simulink model "single_phase_ttype_inverter"  (R2026a)
settings: Solver=ode23tb  StopTime=simlength  FixedStep=tc  MaxStep=glb_time.tc
values from neighbouring files (symbols this model uses):
  afe_ctrl = param.afe.ctrl    [init_model.m]
  afe_pwm_phase_shift_mod1 = param.afe.behav.pwm_phase_shift_mod1    [init_model.m]
  DThs_init = param.thermal.DThs_init    [init_model.m]
  filters = param.ctrl.filters    [init_model.m]
  frt_data = param.frt.data    [init_model.m]
  glb_time = param.glb_time    [init_model.m]
  grid_emu = param.grid.emu    [init_model.m]
  kepsilon = param.spinv.kepsilon    [init_model.m]
  kp_align = param.ctrl.kp_align    [init_model.m]
  lim_down_align = param.ctrl.lim_down_align    [init_model.m]
  lim_up_align = param.ctrl.lim_up_align    [init_model.m]
  mavarage_filter_frequency_base_order = param.ctrl.mavarage_filter_frequency_base_order    [init_model.m]
  omega_set = param.spinv.omega_set    [init_model.m]
  single_phase_inverter_ctrl = param.spinv.ctrl    [init_model.m]
  Tambient = param.thermal.Tambient    [init_model.m]
  time_aux_power_supply_fault = param.sim.time_aux_power_supply_fault    [init_model.m]
  time_step_ref_1 = param.spinv.ref.time_step_ref_1    [init_model.m]
  time_step_ref_2 = param.spinv.ref.time_step_ref_2    [init_model.m]
  time_step_ref_3 = param.spinv.ref.time_step_ref_3    [init_model.m]
undefined symbols (not defined in the file or in its folder): delta_fht1, hwdata, ki_align, Ld_fht1, magnitude, omega_fht1, ts_inv, Vac_FS, Vdc_nom, Xbez
libraries: fl_lib x61, nesl_utility x39, moving_average_filter x11, moving_average_filter_cc x8, discrete_time_low_pass_filter x4, sl_discontinuities x3, single_phase_transformer_lib x3, linear_double_integrator_observer_ccaller x2, phase_shift_filter_ccaller x2, threephase_inductor_lib x1, dclink_for_two_levels x1, three_phase_pwm_modulator x1
(part 3 of 9)

== system single_phase_ttype_inverter/single_phase_inverter/single phase inverter control/acquisition_and_scaling_grid_voltage_ac ==
  in : Inport
  1/Ti5 : Gain  Gain=1/grid_emu.u2bez  SaturateOnIntegerOverflow=on  OutDataTypeStr=Inherit: Same as input  ParamDataTypeStr=Inherit: Same as input
  Quantizer : Quantizer  QuantizationInterval=adc12_quantization
  out : Outport
  wires:
  Quantizer/1 -> out/1
  1/Ti5/1 -> Quantizer/1
  in/1 -> 1/Ti5/1

== system single_phase_ttype_inverter/single_phase_inverter/single phase inverter control/acquisition_and_scaling_voltage ==
  in : Inport
  1/Ti5 : Gain  Gain=1/hwdata.single_phase_inverter.ubez  SaturateOnIntegerOverflow=on  OutDataTypeStr=Inherit: Same as input  ParamDataTypeStr=Inherit: Same as input
  Quantizer : Quantizer  QuantizationInterval=adc12_quantization
  pwm filtering for measure : cstblocks_lti/LTI System  sys=sogi.flt.beta  IC=[]  PadeOrder=0
  out : Outport
  wires:
  in/1 -> 1/Ti5/1
  pwm filtering for measure/1 -> Quantizer/1
  1/Ti5/1 -> pwm filtering for measure/1
  Quantizer/1 -> out/1

== system single_phase_ttype_inverter/single_phase_inverter/single phase inverter control/inverter_current_output_pu_reference ==
  Gain : Gain
  Rate Limiter : RateLimiter  RisingSlewLimit=hwdata.single_phase_inverter.ibez  FallingSlewLimit=-hwdata.single_phase_inverter.ibez  SampleTimeMode=inherited
  Sum : Sum  Inputs=+++
  i_out_inverter_reference_step1 : Step  Time=time_step_ref_1  FinalValue=iph_grid_pu_ref_1  SampleTime=0
  i_out_inverter_reference_step2 : Step  Time=time_step_ref_2  FinalValue=iph_grid_pu_ref_2  SampleTime=0
  i_out_inverter_reference_step3 : Step  Time=time_step_ref_3  FinalValue=iph_grid_pu_ref_3  SampleTime=0
  inverter_current_output_pu_reference : Outport
  wires:
  Rate Limiter/1 -> Gain/1
  Sum/1 -> Rate Limiter/1
  Gain/1 -> inverter_current_output_pu_reference/1
  i_out_inverter_reference_step1/1 -> Sum/2
  i_out_inverter_reference_step2/1 -> Sum/3
  i_out_inverter_reference_step3/1 -> Sum/1

== system single_phase_ttype_inverter/single_phase_inverter/single phase inverter control/pwm modulator ==
  vout : Inport
  Constant : Constant  Value=0
  single_phase_three_levels_PWM_generator_with_global_TRGO : single_phase_three_levels_PWM_modulator/single_phase_three_levels_PWM_generator_with_global_TRGO  f=glb_time.fPWM_INV  m_up=1  m_low=-1  dead_time=glb_time.dead_time_INV  pos_cmd_gate=15  neg_cmd_gate=-10  polarity=1  tc=glb_time.tc  double_sampling=0
  gate_cmds : Outport
  tag scope: TRGO_INV_1=global
  wires:
  vout/1 -> single_phase_three_levels_PWM_generator_with_global_TRGO/3
  Constant/1 -> single_phase_three_levels_PWM_generator_with_global_TRGO/2
  single_phase_three_levels_PWM_generator_with_global_TRGO/2 -> gate_cmds/1
  single_phase_three_levels_PWM_generator_with_global_TRGO/1 -> [TRGO_INV_1]
  [local_time_inverter] -> single_phase_three_levels_PWM_generator_with_global_TRGO/1

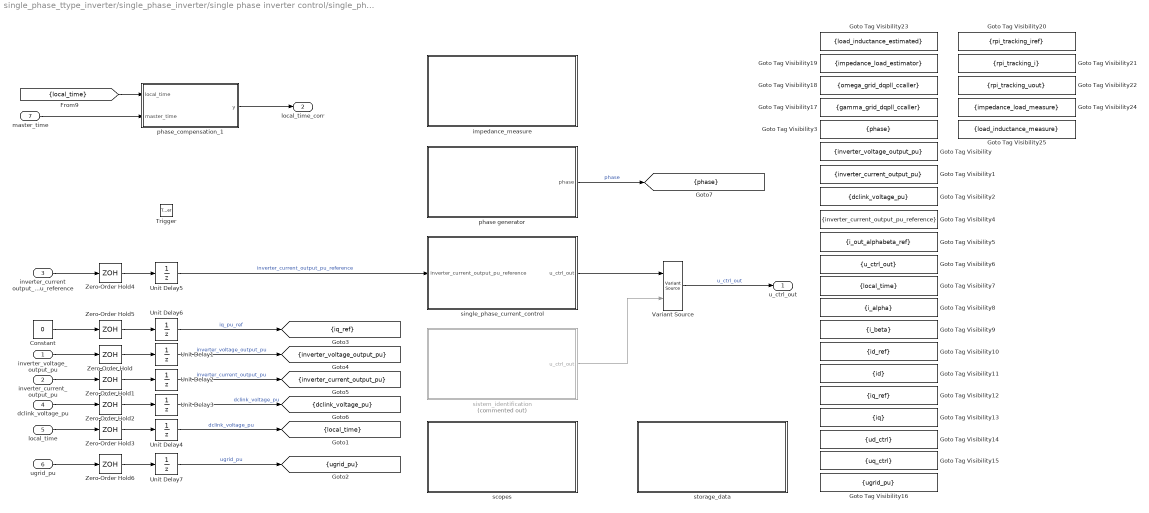
== system single_phase_ttype_inverter/single_phase_inverter/single phase inverter control/single_phase_inverter_ctrl ==
  inverter_voltage_output_pu : Inport
  inverter_current_output_pu : Inport  Port=2
  inverter_current output_pu_reference : Inport  Port=3
  dclink_voltage_pu : Inport  Port=4
  local_time : Inport  Port=5
  ugrid_pu : Inport  Port=6
  master_time : Inport  Port=7
  Trigger : TriggerPort  VariantControl=(inherit)  PortDimensions=1
  Constant : Constant  Value=0
  Goto Tag Visibility : GotoTagVisibility  GotoTag=inverter_voltage_output_pu
  Goto Tag Visibility1 : GotoTagVisibility  GotoTag=inverter_current_output_pu
  Goto Tag Visibility10 : GotoTagVisibility  GotoTag=id_ref
  Goto Tag Visibility11 : GotoTagVisibility  GotoTag=id
  Goto Tag Visibility12 : GotoTagVisibility  GotoTag=iq_ref
  Goto Tag Visibility13 : GotoTagVisibility  GotoTag=iq
  Goto Tag Visibility14 : GotoTagVisibility  GotoTag=ud_ctrl
  Goto Tag Visibility15 : GotoTagVisibility  GotoTag=uq_ctrl
  Goto Tag Visibility16 : GotoTagVisibility  GotoTag=ugrid_pu
  Goto Tag Visibility17 : GotoTagVisibility  GotoTag=gamma_grid_dqpll_ccaller
  Goto Tag Visibility18 : GotoTagVisibility  GotoTag=omega_grid_dqpll_ccaller
  Goto Tag Visibility19 : GotoTagVisibility  GotoTag=impedance_load_estimator
  Goto Tag Visibility2 : GotoTagVisibility  GotoTag=dclink_voltage_pu
  Goto Tag Visibility20 : GotoTagVisibility  GotoTag=rpi_tracking_iref
  Goto Tag Visibility21 : GotoTagVisibility  GotoTag=rpi_tracking_i
  Goto Tag Visibility22 : GotoTagVisibility  GotoTag=rpi_tracking_uout
  Goto Tag Visibility23 : GotoTagVisibility  GotoTag=load_inductance_estimated
  Goto Tag Visibility24 : GotoTagVisibility  GotoTag=impedance_load_measure
  Goto Tag Visibility25 : GotoTagVisibility  GotoTag=load_inductance_measure
  Goto Tag Visibility3 : GotoTagVisibility  GotoTag=phase
  Goto Tag Visibility4 : GotoTagVisibility  GotoTag=inverter_current_output_pu_reference
  Goto Tag Visibility5 : GotoTagVisibility  GotoTag=i_out_alphabeta_ref
  Goto Tag Visibility6 : GotoTagVisibility  GotoTag=u_ctrl_out
  Goto Tag Visibility7 : GotoTagVisibility  GotoTag=local_time
  Goto Tag Visibility8 : GotoTagVisibility  GotoTag=i_alpha
  Goto Tag Visibility9 : GotoTagVisibility  GotoTag=i_beta
  Unit Delay{1..7} (7 alike) : UnitDelay  SampleTime=-1
  Variant Source : VariantSource  VariantControls={system_identification_enable == 0, system_identification_enable == 1}
  Zero-Order Hold{,1..6} (7 alike) : ZeroOrderHold  SampleTime=-1
  impedance_measure : Subsystem
  phase generator : Subsystem
  phase_compensation_1 : Subsystem
  scopes : Subsystem
  single_phase_current_control : Subsystem
  sistem_identification : Subsystem  Commented=on
  storage_data : Subsystem
  u_ctrl_out : Outport
  local_time_corr : Outport  Port=2
  tag scope: dclink_voltage_pu=scoped, inverter_current_output_pu=scoped, inverter_voltage_output_pu=scoped, iq_ref=scoped, local_time=scoped, phase=scoped, ugrid_pu=scoped
  wires:
  inverter_voltage_output_pu/1 -> Zero-Order Hold/1
  inverter_current_output_pu/1 -> Zero-Order Hold1/1
  dclink_voltage_pu/1 -> Zero-Order Hold2/1
  Unit Delay1/1 -> [inverter_voltage_output_pu]  "inverter_voltage_output_pu"
  Unit Delay2/1 -> [inverter_current_output_pu]  "inverter_current_output_pu"
  Unit Delay3/1 -> [dclink_voltage_pu]  "dclink_voltage_pu"
  phase generator/1(phase) -> [phase]  "phase"
  inverter_current output_pu_reference/1 -> Zero-Order Hold4/1
  single_phase_current_control/1(u_ctrl_out) -> Variant Source/1
  Variant Source/1 -> u_ctrl_out/1  "u_ctrl_out"
  sistem_identification/1(u_ctrl_out) -> Variant Source/2
  Zero-Order Hold/1 -> Unit Delay1/1
  Zero-Order Hold1/1 -> Unit Delay2/1
  Zero-Order Hold2/1 -> Unit Delay3/1
  Zero-Order Hold3/1 -> Unit Delay4/1
  Unit Delay4/1 -> [local_time]  "dclink_voltage_pu"
  local_time/1 -> Zero-Order Hold3/1
  Zero-Order Hold4/1 -> Unit Delay5/1
  Unit Delay5/1 -> single_phase_current_control/1(inverter_current_output_pu_reference)  "inverter_current_output_pu_reference"
  Constant/1 -> Zero-Order Hold5/1
  Zero-Order Hold5/1 -> Unit Delay6/1
  Unit Delay6/1 -> [iq_ref]  "iq_pu_ref"
  ugrid_pu/1 -> Zero-Order Hold6/1
  Zero-Order Hold6/1 -> Unit Delay7/1
  Unit Delay7/1 -> [ugrid_pu]  "ugrid_pu"
  [local_time] -> phase_compensation_1/1(local_time)
  phase_compensation_1/1(y) -> local_time_corr/1
  master_time/1 -> phase_compensation_1/2(master_time)

== system single_phase_ttype_inverter/afe/AFE_control/afe_control/FRT-VDE4110 ==
  FRT-Detection : Subsystem
  FRT-PosNegReactiveCurrentReferences : Subsystem
  frt_detection_output : Scope  NumInputPorts=3
      settings: ActiveDisplayYMinimum=-0.12499999999999997  ActiveDisplayYMaximum=1.125
  tag scope: frt_active_mod1=global, pwr_lim_enable_mod1=global
  wires:
  [v_grid_pos_xi_avg_mod1] -> FRT-PosNegReactiveCurrentReferences/1(In1)
  [v_grid_neg_xi_avg_mod1] -> FRT-PosNegReactiveCurrentReferences/3(In3)
  [v_grid_neg_eta_avg_mod1] -> FRT-PosNegReactiveCurrentReferences/4(In4)
  [v_grid_pos_eta_avg_mod1] -> FRT-PosNegReactiveCurrentReferences/2(In2)
  FRT-Detection/4(frt_active) -> frt_detection_output/2, [frt_active_mod1]  "frt_active"
  FRT-Detection/5(pwr_lim_enable) -> frt_detection_output/3, [pwr_lim_enable_mod1]  "pwr_lim_enable"
  FRT-Detection/2(frt_state) -> frt_detection_output/1  "frt_state"

== system single_phase_ttype_inverter/afe/AFE_control/afe_control/current_ctrl ==
  i_xi_ref : Inport
  Demux : Demux  Outputs=3
  current_transformation : Subsystem
  inner_current_ctrl : Subsystem
  xieta2abc : Subsystem
  uab_out : Outport
  wires:
  Demux/1 -> current_transformation/1(is_a_pu)  "is_a"
  Demux/2 -> current_transformation/2(is_b_pu)  "is_b"
  Demux/3 -> current_transformation/3(is_c_pu)  "is_c"
  [isd_abc_pu_mod1] -> Demux/1
  [phase_grid_pll_mod1] -> xieta2abc/5(phase)
  xieta2abc/1(i_abc) -> inner_current_ctrl/1(In1)
  [isd_abc_pu_mod1] -> inner_current_ctrl/2(is_abc)
  inner_current_ctrl/1(uab) -> uab_out/1
  i_xi_ref/1 -> xieta2abc/1(pos_xi)  "i_xi_ref"
  [i_stack_neg_eta_ref_mod1] -> xieta2abc/4(neg_eta)
  [i_stack_neg_xi_ref_mod1] -> xieta2abc/3(neg_xi)
  [i_stack_pos_eta_ref_mod1] -> xieta2abc/2(pos_eta)

== system single_phase_ttype_inverter/afe/AFE_control/afe_control/data_to_worspace_module_1 ==
  Bus Selector : BusSelector  OutputSignals=i_grid_pos_eta_ref,i_grid_neg_eta_ref,i_grid_neg_xi_ref
  To Workspace1 : ToWorkspace  VariableName=i_grid_pos_eta_ref_sim_mod1  SampleTime=-1
      settings: MaxDataPoints=glb_time.Ns_afe
  To Workspace11 : ToWorkspace  VariableName=i_grid_pos_xi_sim_mod1  SampleTime=-1
      settings: MaxDataPoints=glb_time.Ns_afe
  To Workspace13 : ToWorkspace  VariableName=i_grid_pos_eta_sim_mod1  SampleTime=-1
      settings: MaxDataPoints=glb_time.Ns_afe
  To Workspace14 : ToWorkspace  VariableName=i_grid_neg_xi_sim_mod1  SampleTime=-1
      settings: MaxDataPoints=glb_time.Ns_afe
  To Workspace15 : ToWorkspace  VariableName=i_grid_neg_eta_sim_mod1  SampleTime=-1
      settings: MaxDataPoints=glb_time.Ns_afe
  To Workspace16 : ToWorkspace  VariableName=u_grid_pos_xi_sim_mod1  SampleTime=-1
      settings: MaxDataPoints=glb_time.Ns_afe
  To Workspace17 : ToWorkspace  VariableName=u_grid_pos_eta_sim_mod1  SampleTime=-1
      settings: MaxDataPoints=glb_time.Ns_afe
  To Workspace18 : ToWorkspace  VariableName=u_grid_neg_xi_sim_mod1  SampleTime=-1
      settings: MaxDataPoints=glb_time.Ns_afe
  To Workspace19 : ToWorkspace  VariableName=u_grid_neg_eta_sim_mod1  SampleTime=-1
      settings: MaxDataPoints=glb_time.Ns_afe
  To Workspace2 : ToWorkspace  VariableName=i_grid_neg_xi_ref_sim_mod1  SampleTime=-1
      settings: MaxDataPoints=glb_time.Ns_afe
  To Workspace3 : ToWorkspace  VariableName=i_grid_neg_eta_ref_sim_mod1  SampleTime=-1
      settings: MaxDataPoints=glb_time.Ns_afe
  wires:
  [i_grid_pos_eta_avg_mod1] -> To Workspace13/1
  [i_grid_pos_xi_avg_mod1] -> To Workspace11/1
  [i_grid_neg_xi_avg_mod1] -> To Workspace14/1
  [i_grid_neg_eta_avg_mod1] -> To Workspace15/1
  [v_grid_pos_xi_avg_mod1] -> To Workspace16/1
  [v_grid_neg_eta_avg_mod1] -> To Workspace19/1
  [v_grid_pos_eta_avg_mod1] -> To Workspace17/1
  [v_grid_neg_xi_avg_mod1] -> To Workspace18/1
  [i_grid_seq_ref_mod1] -> Bus Selector/1
  Bus Selector/1 -> To Workspace1/1  "<i_grid_pos_eta_ref>"
  Bus Selector/2 -> To Workspace3/1  "<i_grid_neg_eta_ref>"
  Bus Selector/3 -> To Workspace2/1  "<i_grid_neg_xi_ref>"

== system single_phase_ttype_inverter/afe/AFE_control/afe_control/grid_current_sequences_and_reactive_pwr_ctrl ==
  ig_abc_pu : Inport
  current_sequence_avg : Subsystem
  grid_current_sampling_and_alpha_beta_transformation : Subsystem
  i_alphabeta2xieta : Subsystem
  sequences_current_control : Subsystem
  tag scope: i_grid_neg_eta_avg_mod1=scoped, i_grid_neg_xi_avg_mod1=scoped, i_grid_pos_eta_avg_mod1=scoped, i_grid_pos_xi_avg_mod1=scoped
  wires:
  i_alphabeta2xieta/1(xi) -> current_sequence_avg/1(i_grid_pos_xi)
  i_alphabeta2xieta/3(v_grid_neg_xi) -> current_sequence_avg/3(i_grid_neg_xi)
  i_alphabeta2xieta/4(e) -> current_sequence_avg/4(i_grid_neg_eta)
  current_sequence_avg/4(i_grid_neg_eta_avg) -> sequences_current_control/4(i_neg_eta), [i_grid_neg_eta_avg_mod1]
  ig_abc_pu/1 -> grid_current_sampling_and_alpha_beta_transformation/1(ig_abc)
  i_alphabeta2xieta/2(v_grid_pos_eta) -> current_sequence_avg/2(i_grid_pos_eta)
  current_sequence_avg/1(i_grid_pos_xi_avg) -> [i_grid_pos_xi_avg_mod1], sequences_current_control/1(i_pos_xi)
  current_sequence_avg/2(i_grid_pos_eta_avg) -> [i_grid_pos_eta_avg_mod1], sequences_current_control/2(i_pos_eta)
  [phase_grid_pll_mod1] -> i_alphabeta2xieta/3(gamma)
  grid_current_sampling_and_alpha_beta_transformation/2(i_grid_beta) -> i_alphabeta2xieta/2(beta)
  grid_current_sampling_and_alpha_beta_transformation/1(i_grid_alpha) -> i_alphabeta2xieta/1(alpha)
  current_sequence_avg/3(i_grid_neg_xi_avg) -> sequences_current_control/3(i_neg_xi), [i_grid_neg_xi_avg_mod1]

== system single_phase_ttype_inverter/afe/AFE_control/afe_control/grid_phase_acquisition ==
  grid_phase : Inport
  Quantizer : Quantizer  QuantizationInterval=adc_quantization
  Unit Delay : UnitDelay  SampleTime=-1
  Zero-Order Hold : ZeroOrderHold  SampleTime=-1
  grid_phased : Outport
  wires:
  Zero-Order Hold/1 -> Quantizer/1
  Unit Delay/1 -> grid_phased/1
  grid_phase/1 -> Zero-Order Hold/1
  Quantizer/1 -> Unit Delay/1

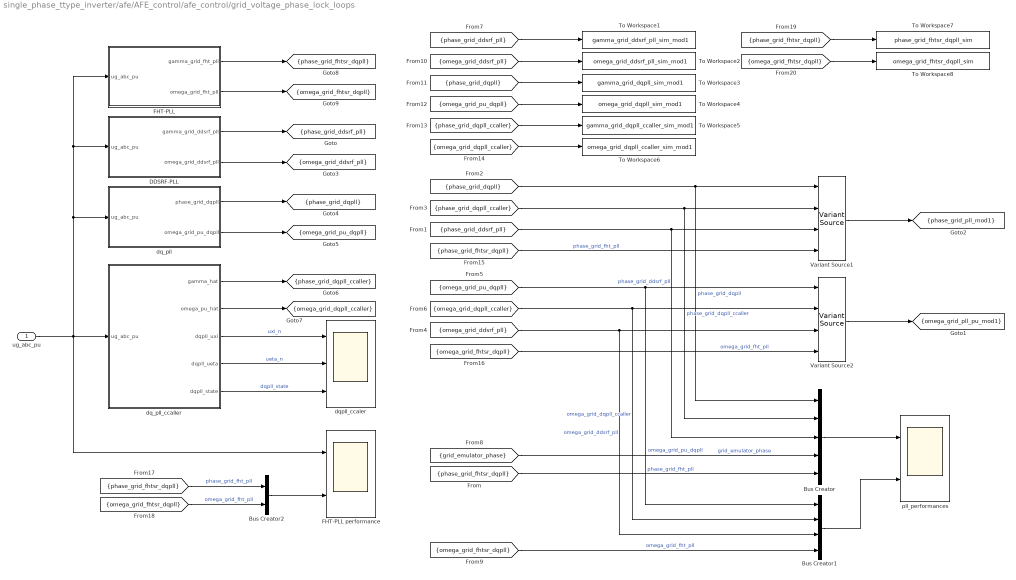
== system single_phase_ttype_inverter/afe/AFE_control/afe_control/grid_voltage_phase_lock_loops ==
  ug_abc_pu : Inport
  Bus Creator : BusCreator  Inputs=5
  Bus Creator1 : BusCreator  Inputs=4
  Bus Creator2 : BusCreator  Inputs=2
  DDSRF-PLL : Subsystem
  FHT-PLL : Subsystem
  FHT-PLL performance : Scope  NumInputPorts=2
      settings: ActiveDisplayYMinimum=-1.251220703125  ActiveDisplayYMaximum=1.251220703125  DataLoggingVariableName=ScopeData8
  To Workspace1 : ToWorkspace  VariableName=gamma_grid_ddsrf_pll_sim_mod1  SampleTime=-1
      settings: MaxDataPoints=glb_time.Ns_afe
  To Workspace2 : ToWorkspace  VariableName=omega_grid_ddsrf_pll_sim_mod1  SampleTime=-1
      settings: MaxDataPoints=glb_time.Ns_afe
  To Workspace3 : ToWorkspace  VariableName=gamma_grid_dqpll_sim_mod1  SampleTime=-1
      settings: MaxDataPoints=glb_time.Ns_afe
  To Workspace4 : ToWorkspace  VariableName=omega_grid_dqpll_sim_mod1  SampleTime=-1
      settings: MaxDataPoints=glb_time.Ns_afe
  To Workspace5 : ToWorkspace  VariableName=gamma_grid_dqpll_ccaller_sim_mod1  SampleTime=-1
      settings: MaxDataPoints=glb_time.Ns_afe
  To Workspace6 : ToWorkspace  VariableName=omega_grid_dqpll_ccaller_sim_mod1  SampleTime=-1
      settings: MaxDataPoints=glb_time.Ns_afe
  To Workspace7 : ToWorkspace  VariableName=phase_grid_fhtsr_dqpll_sim  SampleTime=-1
      settings: MaxDataPoints=glb_time.Ns_afe
  To Workspace8 : ToWorkspace  VariableName=omega_grid_fhtsr_dqpll_sim  SampleTime=-1
      settings: MaxDataPoints=glb_time.Ns_afe
  Variant Source1 : VariantSource  VariantControls={use_dq_pll_mode1 == 1, use_dq_pll_mode2 == 1, use_dq_pll_mode3 == 1, use_dq_pll_mode4 == 1}
  Variant Source2 : VariantSource  VariantControls={use_dq_pll_mode1 == 1, use_dq_pll_mode2 == 1, use_dq_pll_mode3 == 1, use_dq_pll_mode4 == 1}
  dq_pll : Subsystem
  dq_pll_ccaller : Subsystem
  dqpll_ccaler : Scope  NumInputPorts=3
      settings: ActiveDisplayYMinimum=-0.88802937790751446  ActiveDisplayYMaximum=4.5431143753230572  DataLoggingVariableName=ScopeData4
  pll_performances : Scope  NumInputPorts=2
      settings: ActiveDisplayYMinimum=-3.922337429985399  ActiveDisplayYMaximum=3.9215931778997177  DataLoggingVariableName=ScopeData34
  tag scope: omega_grid_ddsrf_pll=scoped, omega_grid_dqpll_ccaller=scoped, omega_grid_fhtsr_dqpll=scoped, omega_grid_pll_pu_mod1=scoped, omega_grid_pu_dqpll=scoped, phase_grid_ddsrf_pll=scoped, phase_grid_dqpll=scoped, phase_grid_dqpll_ccaller=scoped, phase_grid_fhtsr_dqpll=scoped, phase_grid_pll_mod1=scoped
  wires:
  Variant Source1/1 -> [phase_grid_pll_mod1]
  DDSRF-PLL/1(gamma_grid_ddsrf_pll) -> [phase_grid_ddsrf_pll]
  DDSRF-PLL/2(omega_grid_ddsrf_pll) -> [omega_grid_ddsrf_pll]
  dq_pll/2(omega_grid_pu_dqpll) -> [omega_grid_pu_dqpll]
  dq_pll/1(phase_grid_dqpll) -> [phase_grid_dqpll]
  dq_pll_ccaller/1(gamma_hat) -> [phase_grid_dqpll_ccaller]
  dq_pll_ccaller/2(omega_pu_hat) -> [omega_grid_dqpll_ccaller]
  [phase_grid_dqpll] -> Variant Source1/1, Bus Creator/1  "phase_grid_dqpll"
  [phase_grid_dqpll_ccaller] -> Bus Creator/2, Variant Source1/2  "phase_grid_dqpll_ccaller"
  [phase_grid_ddsrf_pll] -> Bus Creator/3, Variant Source1/3  "phase_grid_ddsrf_pll"
  [omega_grid_pu_dqpll] -> Variant Source2/1, Bus Creator1/1  "omega_grid_pu_dqpll"
  [omega_grid_dqpll_ccaller] -> Variant Source2/2, Bus Creator1/2  "omega_grid_dqpll_ccaller"
  [omega_grid_ddsrf_pll] -> Variant Source2/3, Bus Creator1/3  "omega_grid_ddsrf_pll"
  Variant Source2/1 -> [omega_grid_pll_pu_mod1]
  dq_pll_ccaller/3(dqpll_uxi) -> dqpll_ccaler/1  "uxi_n"
  dq_pll_ccaller/4(dqpll_ueta) -> dqpll_ccaler/2  "ueta_n"
  dq_pll_ccaller/5(dqpll_state) -> dqpll_ccaler/3  "dqpll_state"
  ug_abc_pu/1 -> FHT-PLL performance/1, dq_pll/1(ug_abc_pu), DDSRF-PLL/1(ug_abc_pu), FHT-PLL/1(ug_abc_pu), dq_pll_ccaller/1(ug_abc_pu)
  [phase_grid_ddsrf_pll] -> To Workspace1/1
  [omega_grid_ddsrf_pll] -> To Workspace2/1
  [phase_grid_dqpll] -> To Workspace3/1
  [omega_grid_pu_dqpll] -> To Workspace4/1
  [phase_grid_dqpll_ccaller] -> To Workspace5/1
  [omega_grid_dqpll_ccaller] -> To Workspace6/1
  Bus Creator/1 -> pll_performances/1
  Bus Creator1/1 -> pll_performances/2
  [grid_emulator_phase] -> Bus Creator/4  "grid_emulator_phase"
  FHT-PLL/2(omega_grid_fht_pll) -> [omega_grid_fhtsr_dqpll]
  FHT-PLL/1(gamma_grid_fht_pll) -> [phase_grid_fhtsr_dqpll]
  [phase_grid_fhtsr_dqpll] -> Bus Creator/5  "phase_grid_fht_pll"
  [omega_grid_fhtsr_dqpll] -> Bus Creator1/4  "omega_grid_fht_pll"
  [phase_grid_fhtsr_dqpll] -> Variant Source1/4  "phase_grid_fht_pll"
  [omega_grid_fhtsr_dqpll] -> Variant Source2/4  "omega_grid_fht_pll"
  Bus Creator2/1 -> FHT-PLL performance/2
  [omega_grid_fhtsr_dqpll] -> Bus Creator2/2  "omega_grid_fht_pll"
  [phase_grid_fhtsr_dqpll] -> Bus Creator2/1  "phase_grid_fht_pll"
  [phase_grid_fhtsr_dqpll] -> To Workspace7/1
  [omega_grid_fhtsr_dqpll] -> To Workspace8/1

== system single_phase_ttype_inverter/afe/AFE_control/afe_control/grid_voltage_sequences ==
  grid_voltage_sampling_and_alpha_beta_transformation : Subsystem
  v_alphabeta2xieta : Subsystem
  voltage_sequence_avg : Subsystem
  tag scope: ug_alpha_pu_mod1=scoped, ug_beta_pu_mod1=scoped, v_grid_neg_eta_avg_mod1=scoped, v_grid_neg_xi_avg_mod1=scoped, v_grid_pos_eta_avg_mod1=scoped, v_grid_pos_xi_avg_mod1=scoped
  wires:
  v_alphabeta2xieta/4(v_grid_neg_eta) -> voltage_sequence_avg/4(v_grid_neg_eta)  "neg_eta"
  v_alphabeta2xieta/2(eta) -> voltage_sequence_avg/2(v_grid_pos_eta)  "pos_eta"
  [phase_grid_pll_mod1] -> v_alphabeta2xieta/3(gamma)
  v_alphabeta2xieta/3(v_grid_neg_xi) -> voltage_sequence_avg/3(v_grid_neg_xi)  "neg_xi"
  voltage_sequence_avg/3(v_grid_neg_xi_avg) -> [v_grid_neg_xi_avg_mod1]
  voltage_sequence_avg/2(v_grid_pos_eta_avg) -> [v_grid_pos_eta_avg_mod1]
  voltage_sequence_avg/4(v_grid_neg_eta_avg) -> [v_grid_neg_eta_avg_mod1]
  grid_voltage_sampling_and_alpha_beta_transformation/2(u_grid_beta) -> [ug_beta_pu_mod1], v_alphabeta2xieta/2(beta)
  voltage_sequence_avg/1(v_grid_pos_xi_avg) -> [v_grid_pos_xi_avg_mod1]
  v_alphabeta2xieta/1(xi) -> voltage_sequence_avg/1(v_grid_pos_xi)  "pos_xi"
  grid_voltage_sampling_and_alpha_beta_transformation/1(u_grid_alpha) -> [ug_alpha_pu_mod1], v_alphabeta2xieta/1(alpha)
  [ugd_abc_pu_mod1] -> grid_voltage_sampling_and_alpha_beta_transformation/1(v_abc)

== system single_phase_ttype_inverter/afe/AFE_control/afe_control/ig afe quantizzation and one step delay ==
  ig_abc_pu : Inport
  Demux1 : Demux  Outputs=3
  Mux1 : Mux  Inputs=3
  ig afe quantizzation and one step delay : Subsystem
  igd_abc_pu : Outport
  wires:
  Demux1/1 -> ig afe quantizzation and one step delay/1(ig_u_pu)
  Demux1/2 -> ig afe quantizzation and one step delay/2(ig_v_pu)
  ig_abc_pu/1 -> Demux1/1
  Mux1/1 -> igd_abc_pu/1
  Demux1/3 -> ig afe quantizzation and one step delay/3(ig_w_pu)
  ig afe quantizzation and one step delay/2(igd_v_pu) -> Mux1/2
  ig afe quantizzation and one step delay/1(igd_u_pu) -> Mux1/1
  ig afe quantizzation and one step delay/3(igd_w_pu) -> Mux1/3

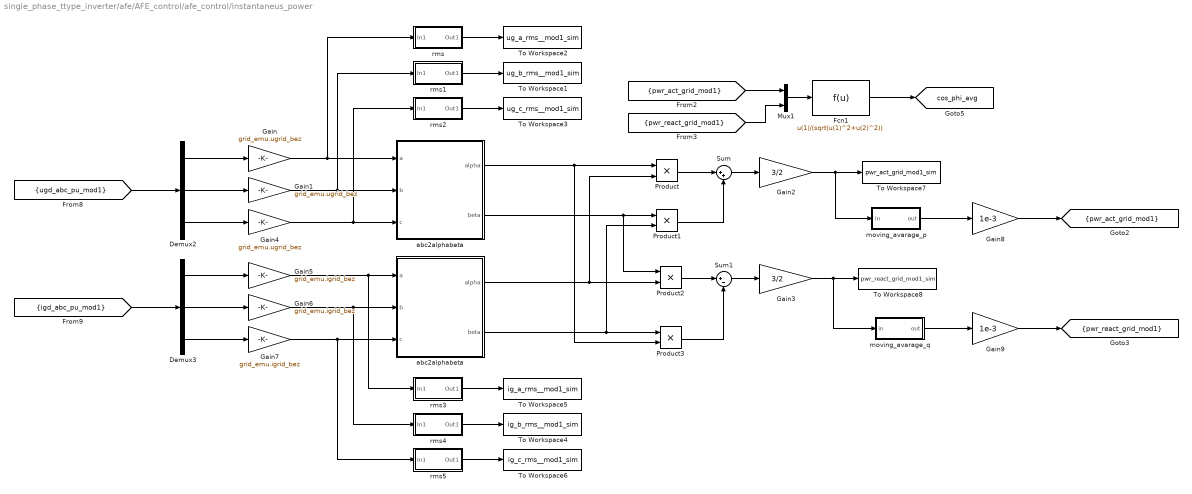
== system single_phase_ttype_inverter/afe/AFE_control/afe_control/instantaneus_power ==
  Demux2 : Demux  Outputs=3
  Demux3 : Demux  Outputs=3
  Fcn1 : Fcn  Expr=u(1)/(sqrt(u(1)^2+u(2)^2))
  Gain : Gain  Gain=grid_emu.ugrid_bez
  Gain1 : Gain  Gain=grid_emu.ugrid_bez
  Gain2 : Gain  Gain=3/2
  Gain3 : Gain  Gain=3/2
  Gain4 : Gain  Gain=grid_emu.ugrid_bez
  Gain5 : Gain  Gain=grid_emu.igrid_bez
  Gain6 : Gain  Gain=grid_emu.igrid_bez
  Gain7 : Gain  Gain=grid_emu.igrid_bez
  Gain8 : Gain  Gain=1e-3
  Gain9 : Gain  Gain=1e-3
  Mux1 : Mux  Inputs=2
  Product{,1..3} (4 alike) : Product  RndMeth=Zero
  Sum : Sum  Inputs=|++
  Sum1 : Sum  Inputs=|+-
  To Workspace1 : ToWorkspace  VariableName=ug_b_rms__mod1_sim  SampleTime=-1
      settings: MaxDataPoints=glb_time.Ns_afe
  To Workspace2 : ToWorkspace  VariableName=ug_a_rms__mod1_sim  SampleTime=-1
      settings: MaxDataPoints=glb_time.Ns_afe
  To Workspace3 : ToWorkspace  VariableName=ug_c_rms__mod1_sim  SampleTime=-1
      settings: MaxDataPoints=glb_time.Ns_afe
  To Workspace4 : ToWorkspace  VariableName=ig_b_rms__mod1_sim  SampleTime=-1
      settings: MaxDataPoints=glb_time.Ns_afe
  To Workspace5 : ToWorkspace  VariableName=ig_a_rms__mod1_sim  SampleTime=-1
      settings: MaxDataPoints=glb_time.Ns_afe
  To Workspace6 : ToWorkspace  VariableName=ig_c_rms__mod1_sim  SampleTime=-1
      settings: MaxDataPoints=glb_time.Ns_afe
  To Workspace7 : ToWorkspace  VariableName=pwr_act_grid_mod1_sim  SampleTime=-1
      settings: MaxDataPoints=glb_time.Ns_afe
  To Workspace8 : ToWorkspace  VariableName=pwr_react_grid_mod1_sim  SampleTime=-1
      settings: MaxDataPoints=glb_time.Ns_afe
  abc2alphabeta : Subsystem
  "abc2alphabeta " : Subsystem
  moving_avarage_p : Subsystem
  moving_avarage_q : Subsystem
  rms : Subsystem
  rms1 : Subsystem
  rms2 : Subsystem
  rms3 : Subsystem
  rms4 : Subsystem
  rms5 : Subsystem
  tag scope: cos_phi_avg=global, pwr_act_grid_mod1=scoped, pwr_react_grid_mod1=scoped
  wires:
  abc2alphabeta/2("beta ") -> Product1/1, Product2/1
  "abc2alphabeta "/2("beta ") -> Product1/2, Product3/1
  abc2alphabeta/1("alpha ") -> Product3/2, Product/1
  "abc2alphabeta "/1("alpha ") -> Product2/2, Product/2
  Product/1 -> Sum/1
  Product1/1 -> Sum/2
  Product2/1 -> Sum1/1
  Product3/1 -> Sum1/2
  Sum1/1 -> Gain3/1
  Sum/1 -> Gain2/1
  Gain2/1 -> moving_avarage_p/1(in), To Workspace7/1
  Gain3/1 -> To Workspace8/1, moving_avarage_q/1(in)
  [pwr_react_grid_mod1] -> Mux1/2
  Mux1/1 -> Fcn1/1
  Fcn1/1 -> [cos_phi_avg]
  [pwr_act_grid_mod1] -> Mux1/1
  rms/1(Out1) -> To Workspace2/1
  rms2/1(Out1) -> To Workspace3/1
  rms1/1(Out1) -> To Workspace1/1
  rms5/1(Out1) -> To Workspace6/1
  rms4/1(Out1) -> To Workspace4/1
  rms3/1(Out1) -> To Workspace5/1
  moving_avarage_p/1(out) -> Gain8/1
  moving_avarage_q/1(out) -> Gain9/1
  Demux2/1 -> Gain/1
  Demux2/2 -> Gain1/1
  Demux2/3 -> Gain4/1
  Demux3/1 -> Gain5/1
  Demux3/2 -> Gain6/1
  Demux3/3 -> Gain7/1
  Gain/1 -> rms/1(In1), abc2alphabeta/1(a)
  Gain1/1 -> rms1/1(In1), abc2alphabeta/2(b)
  Gain4/1 -> rms2/1(In1), abc2alphabeta/3(c)
  Gain5/1 -> rms3/1(In1), "abc2alphabeta "/1(a)
  Gain6/1 -> rms4/1(In1), "abc2alphabeta "/2(b)
  Gain7/1 -> rms5/1(In1), "abc2alphabeta "/3(c)
  Gain8/1 -> [pwr_act_grid_mod1]
  Gain9/1 -> [pwr_react_grid_mod1]
  [ugd_abc_pu_mod1] -> Demux2/1
  [igd_abc_pu_mod1] -> Demux3/1

== system single_phase_ttype_inverter/afe/AFE_control/afe_control/interesting scopes ==
  current_sequences_mod1 : Scope  NumInputPorts=4
      settings: ActiveDisplayYMinimum=-1.4062410671621262  ActiveDisplayYMaximum=0.648263540608363  DataLoggingVariableName=ScopeData2
  i_grid_seq_ref : Scope
      settings: ActiveDisplayYMinimum=-1.125  ActiveDisplayYMaximum=0.125
  voltage_sequences_mod1 : Scope  NumInputPorts=4
      settings: ActiveDisplayYMinimum=-1.2405151816982258  ActiveDisplayYMaximum=1.2605257614333911
  wires:
  [v_grid_neg_eta_avg_mod1] -> voltage_sequences_mod1/4  "u_grid_neg_eta"
  [i_grid_neg_xi_avg_mod1] -> current_sequences_mod1/3  "i_grid_neg_xi"
  [v_grid_pos_eta_avg_mod1] -> voltage_sequences_mod1/2  "u_grid_pos_eta"
  [v_grid_neg_xi_avg_mod1] -> voltage_sequences_mod1/3  "u_grid_neg_xi"
  [i_grid_pos_xi_avg_mod1] -> current_sequences_mod1/1  "i_grid_pos_xi"
  [i_grid_neg_eta_avg_mod1] -> current_sequences_mod1/4  "i_grid_neg_eta"
  [v_grid_pos_xi_avg_mod1] -> voltage_sequences_mod1/1  "u_grid_pos_xi"
  [i_grid_pos_eta_avg_mod1] -> current_sequences_mod1/2  "i_grid_pos_eta"
  [i_grid_seq_ref_mod1] -> i_grid_seq_ref/1  "i_grid_seq_ref"

== system single_phase_ttype_inverter/afe/AFE_control/afe_control/is afe quantizzation and one step delay ==
  is_abc_pu : Inport
  Demux : Demux  Outputs=3
  Mux : Mux  Inputs=3
  is afe quantizzation and one step delay : Subsystem
  isd_abc_pu : Outport
  wires:
  is afe quantizzation and one step delay/2(isd_v_pu) -> Mux/2
  is_abc_pu/1 -> Demux/1
  is afe quantizzation and one step delay/3(isd_w_pu) -> Mux/3
  is afe quantizzation and one step delay/1(isd_u_pu) -> Mux/1
  Demux/1 -> is afe quantizzation and one step delay/1(is_u_pu)
  Mux/1 -> isd_abc_pu/1
  Demux/3 -> is afe quantizzation and one step delay/3(is_w_pu)
  Demux/2 -> is afe quantizzation and one step delay/2(is_v_pu)

== system single_phase_ttype_inverter/afe/AFE_control/afe_control/islanding_mode_detector ==
  gamma : Inport
  alpha : Inport  Port=2
  beta : Inport  Port=3
  Gain : Gain  Gain=7
  MATLAB Function : MATLAB Function  TreatAsAtomicUnit=on
  To Workspace20 : ToWorkspace  VariableName=u_7th_eta_sim_mod1  SampleTime=-1
      settings: MaxDataPoints=glb_time.Ns_afe
  To Workspace21 : ToWorkspace  VariableName=u_7th_xi_sim_mod1  SampleTime=-1
      settings: MaxDataPoints=glb_time.Ns_afe
  bounder : MATLAB Function  TreatAsAtomicUnit=on
  moving_avarage_1 : Subsystem
  moving_avarage_2 : Subsystem
  seventh_ugrid_component : Scope  NumInputPorts=2
      settings: ActiveDisplayYMinimum=-0.0034745064787606167  ActiveDisplayYMaximum=0.0074022094547510631  DataLoggingVariableName=ScopeData10
  tag scope: u_7th_eta_avg_mod1=scoped, u_7th_xi_avg_mod1=scoped
  wires:
  gamma/1 -> Gain/1  "gamma_grid"
  MATLAB Function/1(xi) -> moving_avarage_1/1(u)
  bounder/1(y) -> MATLAB Function/3(gamma)
  Gain/1 -> bounder/1(u)
  alpha/1 -> MATLAB Function/1(alpha)  "u_grid_alpha"
  beta/1 -> MATLAB Function/2(beta)  "u_grid_beta"
  MATLAB Function/2(eta) -> moving_avarage_2/1(u)
  [u_7th_xi_avg_mod1] -> To Workspace21/1
  [u_7th_eta_avg_mod1] -> To Workspace20/1
  moving_avarage_1/1(y) -> [u_7th_xi_avg_mod1], seventh_ugrid_component/1  "u_7th_xi"
  moving_avarage_2/1(y) -> [u_7th_eta_avg_mod1], seventh_ugrid_component/2  "u_7th_eta"

== system single_phase_ttype_inverter/afe/AFE_control/afe_control/phase_compensation_1 ==
  local_time : Inport
  master_time : Inport  Port=2
  Zero-Order Hold : ZeroOrderHold  SampleTime=-1
  Zero-Order Hold1 : ZeroOrderHold  SampleTime=-1
  alignment_eval_afe1 : Subsystem
  y : Outport
  wires:
  local_time/1 -> Zero-Order Hold/1
  master_time/1 -> Zero-Order Hold1/1
  alignment_eval_afe1/1(dp) -> y/1
  Zero-Order Hold/1 -> alignment_eval_afe1/1(local_time)
  Zero-Order Hold1/1 -> alignment_eval_afe1/2(master_time)

== system single_phase_ttype_inverter/afe/AFE_control/afe_control/space_vector ==
  uab_out : Inport
  Bus Creator : BusCreator  Inputs=3
  Bus Selector : BusSelector  OutputSignals=da,db,dc
  Bus Selector1 : BusSelector  OutputSignals=ualpha_afe,ubeta_afe
  C Caller : CCaller  FunctionName=sv_pwm_process_simulink  PortSpecificationStruct="%)30     .    V @   8    (     @         %    \"     4    !     0         %  0 \"0    $    _    07)G3F%M90  4&]R=$YA;64 4V-O<&4     26YD97@     5'EP90      4VEZ90      27-';&]B86P   X    P    !@    @    $          4    (     0    ,    !         !   P!O=70 #@   #     &    \"     0         !0    @    !     P    $         $  # &]U=  .    .     8    (    !          %    \"     $    &     0         0   ...(+2669 chars)"
  Constant : Constant  Value=glb_time.ts_afe
  Constant1 : Constant
  Data Type Conversion1 : DataTypeConversion  OutDataTypeStr=double  SaturateOnIntegerOverflow=off  RndMeth=Floor
  Data Type Conversion15 : DataTypeConversion  OutDataTypeStr=single  SaturateOnIntegerOverflow=off  RndMeth=Floor
  Data Type Conversion16 : DataTypeConversion  OutDataTypeStr=single  SaturateOnIntegerOverflow=off  RndMeth=Floor
  Data Type Conversion17 : DataTypeConversion  OutDataTypeStr=uint32  SaturateOnIntegerOverflow=off  RndMeth=Floor
  Data Type Conversion18 : DataTypeConversion  OutDataTypeStr=single  SaturateOnIntegerOverflow=off  RndMeth=Floor
  Data Type Conversion2 : DataTypeConversion  OutDataTypeStr=double  SaturateOnIntegerOverflow=off  RndMeth=Floor
  Data Type Conversion3 : DataTypeConversion  OutDataTypeStr=double  SaturateOnIntegerOverflow=off  RndMeth=Floor
  Gain1 : Gain  Gain=sqrt(3)/2
  Gain2 : Gain  Gain=sqrt(3)/2
  duvw : Outport
  wires:
  Data Type Conversion15/1 -> C Caller/2
  Bus Selector/2 -> Data Type Conversion2/1  "<db>"
  Data Type Conversion16/1 -> C Caller/3
  Data Type Conversion18/1 -> C Caller/1
  C Caller/1 -> Bus Selector/1
  Bus Creator/1 -> duvw/1
  Data Type Conversion17/1 -> C Caller/4
  Data Type Conversion1/1 -> Bus Creator/1  "du(k)"
  Bus Selector1/2 -> Gain2/1  "<ubeta_afe>"
  Bus Selector/3 -> Data Type Conversion3/1  "<dc>"
  Bus Selector1/1 -> Gain1/1  "<ualpha_afe>"
  Data Type Conversion2/1 -> Bus Creator/2  "dv(k)"
  Gain2/1 -> Data Type Conversion15/1
  Bus Selector/1 -> Data Type Conversion1/1  "<da>"
  Gain1/1 -> Data Type Conversion18/1
  Data Type Conversion3/1 -> Bus Creator/3  "dw(k)"
  Constant/1 -> Data Type Conversion16/1
  uab_out/1 -> Bus Selector1/1
  Constant1/1 -> Data Type Conversion17/1

== system single_phase_ttype_inverter/afe/AFE_control/afe_control/udc_acquisition ==
  udc_pu : Inport
  Quantizer : Quantizer  QuantizationInterval=adc_quantization
  Unit Delay : UnitDelay  SampleTime=-1
  Zero-Order Hold : ZeroOrderHold  SampleTime=-1
  udcd_pu : Outport
  wires:
  Quantizer/1 -> Unit Delay/1
  udc_pu/1 -> Zero-Order Hold/1
  Unit Delay/1 -> udcd_pu/1
  Zero-Order Hold/1 -> Quantizer/1

== system single_phase_ttype_inverter/afe/AFE_control/afe_control/udc_ctrl ==
  udc_pu : Inport
  udc_pu_ref : Inport  Port=2
  1/Ti : Gain  Gain=afe_ctrl.kp_udc_ctrl  SaturateOnIntegerOverflow=on  OutDataTypeStr=Inherit: Same as input  ParamDataTypeStr=Inherit: Same as input
  Constant : Constant  Value=0
  Gain : Gain  Gain=-1
  Saturation : Saturate  UpperLimit=afe_ctrl.ixi_pos_ref_lim  LowerLimit=-afe_ctrl.ixi_pos_ref_lim
  Sum1 : Sum  Inputs=+++  SaturateOnIntegerOverflow=on
  Sum2 : Sum  Inputs=-+  SaturateOnIntegerOverflow=on
  Sum3 : Sum  Inputs=-+  SaturateOnIntegerOverflow=on
  Switch : Switch  Criteria=u2 > Threshold  SaturateOnIntegerOverflow=off  InputSameDT=off
  To Workspace1 : ToWorkspace  VariableName=udc_pu_sim_mod1  SampleTime=-1
      settings: MaxDataPoints=glb_time.Ns_afe
  To Workspace3 : ToWorkspace  VariableName=udc_pu_ref_sim_mod1  SampleTime=-1
      settings: MaxDataPoints=glb_time.Ns_afe
  Unit Delay4 : UnitDelay  SampleTime=-1
  kp : Gain  Gain=afe_ctrl.ki_udc_ctrl*glb_time.ts_afe  SaturateOnIntegerOverflow=on  OutDataTypeStr=Inherit: Same as input  ParamDataTypeStr=Inherit: Same as input
  udc_tracking : Scope  NumInputPorts=2
      settings: ActiveDisplayYMinimum=-0.14752197265624997  ActiveDisplayYMaximum=1.32769775390625  DataLoggingVariableName=ScopeData8
  i_xi_ref : Outport
  wires:
  1/Ti/1 -> Sum1/1, Sum3/1
  kp/1 -> Sum1/2
  Sum3/1 -> Unit Delay4/1
  Unit Delay4/1 -> Sum1/3
  udc_pu_ref/1 -> To Workspace3/1, udc_tracking/1, Sum2/2  "udc_pu_ref"
  udc_pu/1 -> To Workspace1/1, udc_tracking/2, Sum2/1  "udc_pu"
  Sum2/1 -> kp/1, 1/Ti/1
  Sum1/1 -> Saturation/1
  [pwr_lim_enable_mod1] -> Switch/2
  Saturation/1 -> Switch/3
  Switch/1 -> Sum3/2, Gain/1
  Constant/1 -> Switch/1
  Gain/1 -> i_xi_ref/1

== system single_phase_ttype_inverter/afe/AFE_control/afe_control/ug afe quantizzation and one step delay ==
  ug_abc_pu : Inport
  Demux : Demux  Outputs=3
  Mux : Mux  Inputs=3
  ug afe quantizzation and one step delay : Subsystem
  ugd_abc_pu : Outport
  wires:
  ug afe quantizzation and one step delay/2(ugd_v_pu) -> Mux/2
  Demux/2 -> ug afe quantizzation and one step delay/2(ug_v_pu)
  Demux/3 -> ug afe quantizzation and one step delay/3(ug_w_pu)
  ug afe quantizzation and one step delay/1(ugd_u_pu) -> Mux/1
  Demux/1 -> ug afe quantizzation and one step delay/1(ug_u_pu)
  ug_abc_pu/1 -> Demux/1
  ug afe quantizzation and one step delay/3(ugd_w_pu) -> Mux/3
  Mux/1 -> ugd_abc_pu/1

== system single_phase_ttype_inverter/afe/afe/sv_pwm/modulator1 ==
  u : Inport
  v : Inport  Port=2
  w : Inport  Port=3
  phase : Inport  Port=4
  Bus Creator : BusCreator  Inputs=3
  Three phase two level PWM generator with global TRGO : three_phase_pwm_modulator/Three phase two level PWM generator with global TRGO  f=glb_time.fPWM_AFE  m_up=0.98  m_low=0.02  dead_time=glb_time.dead_time_AFE  pos_cmd_gate=15  neg_cmd_gate=-10  polarity=1  tc=glb_time.tc  double_sampling=1
      link override gate commands/Bus Selector: OutputSignals=du(t)
      link override gate commands/Bus Selector1: OutputSignals=dv(t)
      link override gate commands/Bus Selector2: OutputSignals=dw(t)
  gate_cmds : Outport
  tag scope: TRGO_afe_module_1=global
  wires:
  [local_time_afe] -> Three phase two level PWM generator with global TRGO/1
  Bus Creator/1 -> Three phase two level PWM generator with global TRGO/3
  Three phase two level PWM generator with global TRGO/1 -> [TRGO_afe_module_1]
  u/1 -> Bus Creator/1
  v/1 -> Bus Creator/2
  w/1 -> Bus Creator/3
  phase/1 -> Three phase two level PWM generator with global TRGO/2
  Three phase two level PWM generator with global TRGO/2 -> gate_cmds/1

== system single_phase_ttype_inverter/single_phase_inverter/single phase inverter control/single_phase_inverter_ctrl/impedance_measure ==
  Constant : Constant  Value=omega_set
  Gain1 : Gain  Gain=1/omega_set
  Product : Product  Inputs=*/*
  Saturation : Saturate  UpperLimit=inf  LowerLimit=0.05
  Saturation1 : Saturate  UpperLimit=inf  LowerLimit=0.05
  Subsystem : Subsystem
  dclink voltage pu : Scope
      settings: ActiveDisplayYMinimum=-0.17324218749999995  ActiveDisplayYMaximum=2.0591796875  DataLoggingVariableName=ScopeData10
  dmavg_flt : moving_average_filter/dmavg_flt  ts=glb_time.ts_afe  enable_time=0.025
  load_measure : Scope  NumInputPorts=4
      settings: ActiveDisplayYMinimum=-0.057375000356417558  ActiveDisplayYMaximum=0.51637500320775809  DataLoggingVariableName=ScopeData2
  module_iload : Subsystem
  module_uctrl_out : Subsystem
  tag scope: impedance_load_measure=scoped, load_inductance_measure=scoped
  wires:
  module_uctrl_out/1(u_ctrl) -> Product/1
  Saturation/1 -> Product/2
  module_iload/1(iload) -> Saturation/1  "Iload"
  [i_alpha] -> load_measure/3, module_iload/1(i_alpha)  "i_alpha_sogi"
  [i_beta] -> load_measure/4, module_iload/2(i_beta)  "i_beta_sogi"
  [uq_ctrl] -> module_uctrl_out/2(uq_ctrl)
  [ud_ctrl] -> module_uctrl_out/1(ud_ctrl)
  Constant/1 -> dmavg_flt/2
  dmavg_flt/1 -> Gain1/1, load_measure/1, [impedance_load_measure]  "Xload"
  Gain1/1 -> load_measure/2, [load_inductance_measure]  "Lload"
  [dclink_voltage_pu] -> Saturation1/1
  Saturation1/1 -> dclink voltage pu/1, Product/3
  Product/1 -> Subsystem/1(Xload)  "Xload"
  Subsystem/1(Xload1) -> dmavg_flt/1

== system single_phase_ttype_inverter/single_phase_inverter/single phase inverter control/single_phase_inverter_ctrl/phase generator ==
  Bus Creator : BusCreator  Inputs=3
  Bus Creator1 : BusCreator  Inputs=2
  Constant : Constant  Value=omega_set
  Gain : Gain  Gain=glb_time.ts_single_phase_inv
  Sum : Sum  Inputs=|++
  Unit Delay : UnitDelay  SampleTime=-1
  Variant Source : VariantSource  VariantControls={frequency_set ~= grid_emu.fgrid_nom, frequency_set == grid_emu.fgrid_nom}
  bounder1 : MATLAB Function  TreatAsAtomicUnit=on
  dq_pll_ccaller : Subsystem
  dqpll_ccaler : Scope  NumInputPorts=2
      settings: ActiveDisplayYMinimum=-1.624956414103508  ActiveDisplayYMaximum=4.624995157122612  DataLoggingVariableName=ScopeData3
  phase : Outport
  tag scope: gamma_grid_dqpll_ccaller=scoped, omega_grid_dqpll_ccaller=scoped
  wires:
  Sum/1 -> Unit Delay/1
  Constant/1 -> Gain/1
  Unit Delay/1 -> bounder1/1(u)
  Gain/1 -> Sum/1
  bounder1/1(y) -> Sum/2, Variant Source/1  "phase"
  dq_pll_ccaller/4(dqpll_ueta) -> Bus Creator/2  "ueta_n"
  dq_pll_ccaller/3(dqpll_uxi) -> Bus Creator/1  "uxi_n"
  dq_pll_ccaller/1(gamma_hat) -> [gamma_grid_dqpll_ccaller]
  dq_pll_ccaller/2(omega_pu_hat) -> [omega_grid_dqpll_ccaller]
  dq_pll_ccaller/5(dqpll_state) -> Bus Creator/3  "dqpll_state"
  [ugrid_pu] -> dq_pll_ccaller/1(ug_abc_pu)
  [gamma_grid_dqpll_ccaller] -> Variant Source/2
  [gamma_grid_dqpll_ccaller] -> Bus Creator1/1  "gamma_grid_dqpll"
  [omega_grid_dqpll_ccaller] -> Bus Creator1/2  "omega_grid_dqpll"
  Bus Creator1/1 -> dqpll_ccaler/2
  Bus Creator/1 -> dqpll_ccaler/1
  Variant Source/1 -> phase/1

== system single_phase_ttype_inverter/single_phase_inverter/single phase inverter control/single_phase_inverter_ctrl/phase_compensation_1 ==
  local_time : Inport
  master_time : Inport  Port=2
  Zero-Order Hold : ZeroOrderHold  SampleTime=-1
  Zero-Order Hold1 : ZeroOrderHold  SampleTime=-1
  alignment_eval_afe1 : Subsystem
  y : Outport
  wires:
  local_time/1 -> Zero-Order Hold/1
  master_time/1 -> Zero-Order Hold1/1
  alignment_eval_afe1/1(dp) -> y/1
  Zero-Order Hold/1 -> alignment_eval_afe1/1(local_time)
  Zero-Order Hold1/1 -> alignment_eval_afe1/2(master_time)

== system single_phase_ttype_inverter/single_phase_inverter/single phase inverter control/single_phase_inverter_ctrl/scopes ==
  Bus Creator1 : BusCreator  Inputs=3
  Bus Creator2 : BusCreator  Inputs=2
  Bus Creator3 : BusCreator  Inputs=2
  Bus Creator4 : BusCreator  Inputs=2
  single phase inverter tracking current scope 1 : Scope  NumInputPorts=2
      settings: ActiveDisplayYMinimum=-2.94378662109375  ActiveDisplayYMaximum=2.91986083984375  DataLoggingVariableName=ScopeData12
  single phase inverter tracking current scope 2 : Scope  NumInputPorts=2
      settings: ActiveDisplayYMinimum=-1.2603759765625  ActiveDisplayYMaximum=1.2652587890625  DataLoggingVariableName=ScopeData2
  wires:
  Bus Creator1/1 -> single phase inverter tracking current scope 1/2  "is_tracking"
  [i_out_alphabeta_ref] -> Bus Creator1/2  "i_out_inverter_pu_ref"
  [inverter_current_output_pu] -> Bus Creator1/3  "inverter_current_output_pu"
  [inverter_voltage_output_pu] -> Bus Creator2/1  "inverter_voltage_output_pu"
  Bus Creator2/1 -> single phase inverter tracking current scope 1/1  "load"
  [inverter_current_output_pu_reference] -> Bus Creator1/1  "inverter_current_output_pu_reference"
  [inverter_current_output_pu] -> Bus Creator2/2  "inverter_current_output_pu"
  [u_ctrl_out] -> Bus Creator3/1  "u_ctrl_out"
  [inverter_voltage_output_pu] -> Bus Creator3/2  "inverter_voltage_output_pu"
  Bus Creator3/1 -> single phase inverter tracking current scope 2/2  "u_load"
  [inverter_current_output_pu] -> Bus Creator4/2  "inverter_current_output_pu"
  [i_out_alphabeta_ref] -> Bus Creator4/1  "i_out_alphabeta_ref"
  Bus Creator4/1 -> single phase inverter tracking current scope 2/1  "i_load"

== system single_phase_ttype_inverter/single_phase_inverter/single phase inverter control/single_phase_inverter_ctrl/single_phase_current_control ==
  inverter_current_output_pu_reference : Inport
  Variant Source : VariantSource  VariantControls={rpi_enable == 1, rpi_enable == 0}
  current_reference_generation : Subsystem
  dqpi_current_controller : Subsystem
  rpi_current_controller : Subsystem
  u_ctrl_out : Outport
  tag scope: i_out_alphabeta_ref=scoped, inverter_current_output_pu_reference=scoped, u_ctrl_out=scoped
  wires:
  rpi_current_controller/1(u_ctrl_out) -> Variant Source/1  "u_ctrl_out"
  dqpi_current_controller/1(u_out) -> Variant Source/2  "u_ctrl_out"
  current_reference_generation/1(is_ref) -> [i_out_alphabeta_ref], rpi_current_controller/1(i_ref)  "i_out_inverter_pu_ref"
  Variant Source/1 -> u_ctrl_out/1, [u_ctrl_out]  "u_ctrl_out"
  [phase] -> current_reference_generation/2(phase)
  inverter_current_output_pu_reference/1 -> current_reference_generation/1(mag_ref), [inverter_current_output_pu_reference]
  current_reference_generation/2(id_ref) -> dqpi_current_controller/1(id_ref)

== system single_phase_ttype_inverter/single_phase_inverter/single phase inverter control/single_phase_inverter_ctrl/sistem_identification ==
  open loop u/f : Subsystem
  u_ctrl_out : Outport
  wires:
  open loop u/f/1(u_out) -> u_ctrl_out/1  "u_ctrl_out"
